simulink model "L2"  (R2023b)
settings: Solver=VariableStepAuto  StartTime=0.0  StopTime=10.0  RelTol=1e-3
libraries: dspsrcs4 x1
settings Model: Creator=vladi  LastModifiedBy=vladi

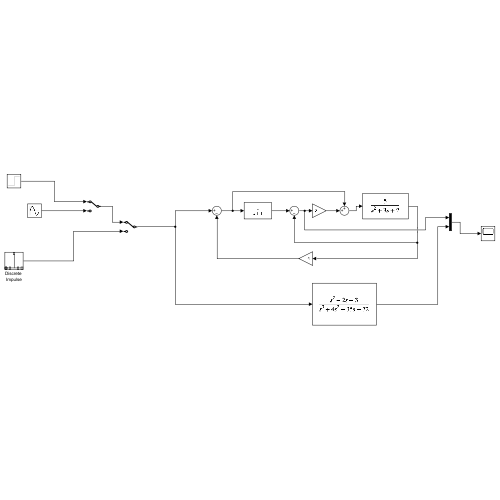
[thumbnail: Simulink's stored preview of the top-level diagram]
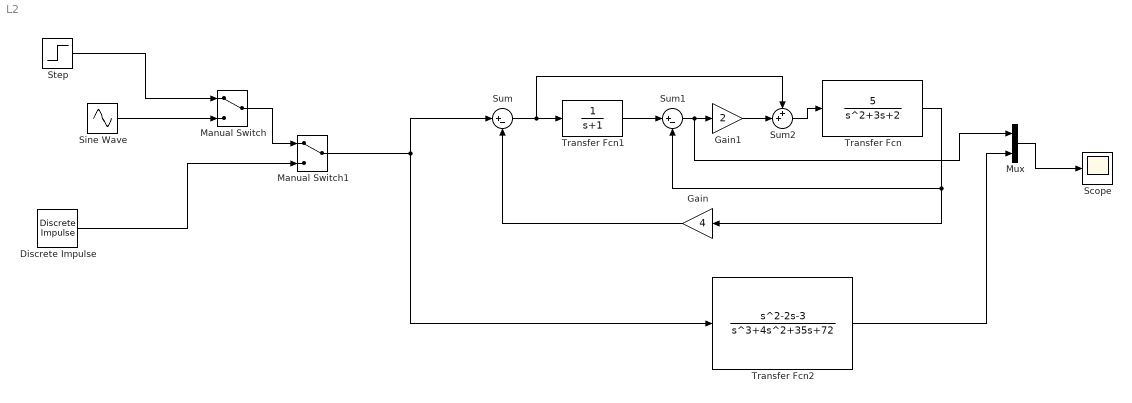
== system L2 ==
  Discrete Impulse : dspsrcs4/Discrete  Impulse  Delay=0  SampleTime=1  FrameSample=1  OutputFrames=off  dataType=double  isSigned=on  wordLen=16  udDataType=sfix(16)  fracBitsMode=Best precision  numFracBits=15  OutDataTypeStr=double  LastOutDataTypeStr=double
  Gain : Gain  Gain=4
  Gain1 : Gain  Gain=2
  Manual Switch : ManualSwitch
  Manual Switch1 : ManualSwitch
  Mux : Mux  Inputs=2
  Scope : Scope
  Sine Wave : Sin  SampleTime=0
  Step : Step  SampleTime=0
  Sum : Sum  Inputs=|+-
  Sum1 : Sum  Inputs=|+-
  Sum2 : Sum  Inputs=++|
  Transfer Fcn : TransferFcn  Numerator=[5]  Denominator=[1 3 2]
  Transfer Fcn1 : TransferFcn  Denominator=[1 1]
  Transfer Fcn2 : TransferFcn  Numerator=[1 -2 -3]  Denominator=[1 4 35 72]
  wires:
  Manual Switch/1 -> Manual Switch1/1
  Manual Switch1/1 -> Sum/1, Transfer Fcn2/1
  Gain/1 -> Sum/2
  Gain1/1 -> Sum2/2
  Step/1 -> Manual Switch/1
  Discrete Impulse/1 -> Manual Switch1/2
  Mux/1 -> Scope/1
  Sum2/1 -> Transfer Fcn/1
  Sum1/1 -> Mux/1, Gain1/1
  Sine Wave/1 -> Manual Switch/2
  Transfer Fcn1/1 -> Sum1/1
  Transfer Fcn2/1 -> Mux/2
  Sum/1 -> Sum2/1, Transfer Fcn1/1
  Transfer Fcn/1 -> Sum1/2, Gain/1
